simulink model "full_sys"  (R2020a)
settings: Solver=VariableStepAuto  StartTime=0.0  StopTime=0.5  RelTol=1e-3
undefined symbols (not defined in the file): Ion, Lithium
libraries: powerlib x22, simulink x2, electricdrivelib x1
settings Model: EnablePacing=on  PacingRate=10  Creator=siddyq  LastModifiedBy=siddyq

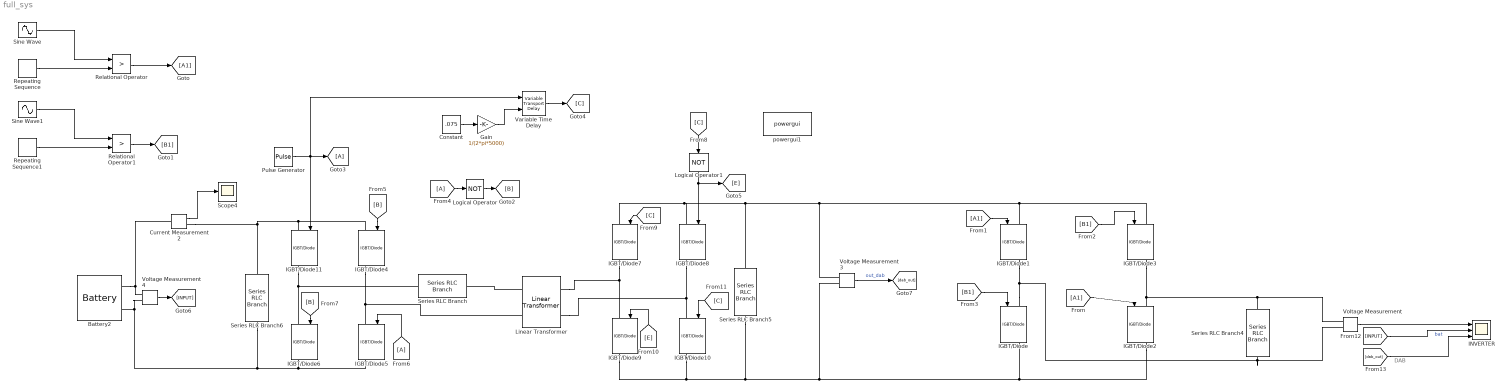
== system full_sys ==
  note: DAB
  Battery2 : electricdrivelib/Extra Sources/Battery  BatType=Lithium-Ion  ShowTempParam=off  ThermalPreset=no  ShowAgeParam=off  NomV=75  NomQ=100  SOC=100  Batt_Tr=1  PresetModel=on  MaxQ=100  MinV=56.25  FullV=87.299  Dis_rate=43.4783  R=0.0075  Normal_OP=90.4348  expZone="[81.0289      4.91304]"  current=[6.5 13 32.5]  Units=Time  Tci=20  NomT=20  T2=-30  MaxQ2=4.8  FullV2=7.1  Normal_OP2=5.655  expZone2="[6.58           1]"  Rca=0.6  ti=2000  Dp=0  Neq0=0  Tsim=1e6  Ta1=25  Qeol=5.4*0.9  Reol=0.013333*1.2  Char_age=[2.3478, 3]  Dis_age=[2.3478, 10]  N1=1500  N2=10500  N3=1000  N4=1400  Ta2=45  N5=950
  Constant : Constant  Value=.075
  Current Measurement2 : powerlib/Measurements/Current Measurement  PhasorSimulation=off  OutputType=Complex  PSBequivalent=0
  Gain : Gain  Gain=1/(2*pi*5000)
  IGBT/Diode{,1..11} (12 alike) : powerlib/Power Electronics/IGBT//Diode  Ron=1e-3  Rs=1e5  Cs=inf  Measurements=on
  INVERTER : Scope  NumInputPorts=3
  Linear Transformer : powerlib/Elements/Linear Transformer  UNITS=SI  NominalPower=[2e2 10000 ]  winding1=[75 0 0]  winding2=[100 0 0]  ThreeWindings=off  winding3=[3.15e+05 66150 42.112]  RmLm=[85555 1.3]  Measurements=None  DataType=on
  Logical Operator : Logic  Operator=NOT  AllPortsSameDT=off  OutDataTypeStr=boolean
  Logical Operator1 : Logic  Operator=NOT  AllPortsSameDT=off  OutDataTypeStr=boolean
  Pulse Generator : DiscretePulseGenerator  PulseType=Time based  Period=1/(2*pi*5000)  PulseWidth=50
  Relational Operator : RelationalOperator  Operator=>  OutDataTypeStr=boolean  RndMeth=Simplest
  Relational Operator1 : RelationalOperator  Operator=>  OutDataTypeStr=boolean  RndMeth=Simplest
  Repeating Sequence : simulink/Sources/Repeating Sequence  rep_seq_t=[0 0.02/40 0.02/20]  rep_seq_y=[0 1 0]
  Repeating Sequence1 : simulink/Sources/Repeating Sequence  rep_seq_t=[0 0.02/40 0.02/20]  rep_seq_y=[0 1 0]
  Scope4 : Scope
  Series RLC Branch : powerlib/Elements/Series RLC Branch  LConnTagsString=__new0  RConnTagsString=__new0  BranchType=L  Resistance=1  Inductance=130e-7  SetiL0=off  InitialCurrent=0  Capacitance=1e-6  Setx0=off  InitialVoltage=0  Measurements=None
  Series RLC Branch4 : powerlib/Elements/Series RLC Branch  LConnTagsString=__new0  RConnTagsString=__new0  BranchType=R  Resistance=10  Inductance=10e-3  SetiL0=off  InitialCurrent=0  Capacitance=1e-6  Setx0=off  InitialVoltage=0  Measurements=None
  Series RLC Branch5 : powerlib/Elements/Series RLC Branch  LConnTagsString=__new0  RConnTagsString=__new0  BranchType=C  Resistance=1  Inductance=1e-3  SetiL0=off  InitialCurrent=0  Capacitance=3000e-6  Setx0=off  InitialVoltage=0  Measurements=None
  Series RLC Branch6 : powerlib/Elements/Series RLC Branch  LConnTagsString=__new0  RConnTagsString=__new0  BranchType=C  Resistance=1  Inductance=1e-3  SetiL0=off  InitialCurrent=0  Capacitance=350e-6  Setx0=off  InitialVoltage=0  Measurements=None
  Sine Wave : Sin  Frequency=100*pi  SampleTime=0
  Sine Wave1 : Sin  Frequency=100*pi  Phase=pi  SampleTime=0
  Variable Time Delay : VariableTransportDelay  MaximumDelay=10  ZeroDelay=on
  Voltage Measurement : powerlib/Measurements/Voltage Measurement  PhasorSimulation=off  OutputType=Complex  PSBequivalent=0
  Voltage Measurement3 : powerlib/Measurements/Voltage Measurement  PhasorSimulation=off  OutputType=Complex  PSBequivalent=0
  Voltage Measurement4 : powerlib/Measurements/Voltage Measurement  PhasorSimulation=off  OutputType=Complex  PSBequivalent=0
  powergui1 : powerlib/powergui  Priority=1  SimulationMode=Discrete  SampleTime=1e-6  frequency=60  Iterations=50  frequencyindice=0  Pbase=100e6  ErrMax=1e-4  UnitsV=kV  UnitsW=MW  buscounter=0  FunctionMessages=off  echomessages=off  EnableUseOfTLC=off  CurrentSourceSwitches=off  DisableSnubberDevices=off  DisableRonSwitches=off  DisableVfSwitches=off  DisplayEquations=off  AutomaticDiscreteSolvers=off  SolverType=Tustin/Backward Euler (TBE)  Interpol=off  ExternalGateDelay=off  methode=off  Ts=100  x0status=blocks  SPID=on  SwTol=0  HookPort=off  NonlinearTolerance=1e-4  nMaxIteration=100  ContinueOnMaxIteration=off  RestoreLinks=warning  ResistiveCurrentMeasurement=off  Frange=[0:2:500]  Ylog=off  Xlog=on  ShowGrid=off  save=off  variable=ZData  structure=0  ZoomFFT=off  StartTime=0.0  cycles=1  DisplayStyle=1  fundamental=60  FreqAxis=off  MaxFrequency=1000  frequencyindicesteady=1  RmsSteady=1  display=off
  wires:
  Relational Operator/1 -> [A1]
  Sine Wave1/1 -> Relational Operator1/1
  Relational Operator1/1 -> [B1]
  Repeating Sequence1/1 -> Relational Operator1/2
  Voltage Measurement/1 -> INVERTER/1
  [A1] -> IGBT/Diode1/1
  [B1] -> IGBT/Diode/1
  [A1] -> IGBT/Diode2/1
  Repeating Sequence/1 -> Relational Operator/2
  Sine Wave/1 -> Relational Operator/1
  [B1] -> IGBT/Diode3/1
  Logical Operator/1 -> [B]
  Voltage Measurement4/1 -> [INPUT]
  [C] -> Logical Operator1/1
  [C] -> IGBT/Diode7/1
  [C] -> IGBT/Diode10/1
  [E] -> IGBT/Diode9/1
  [A] -> IGBT/Diode5/1
  Variable Time Delay/1 -> [C]
  Constant/1 -> Gain/1
  [B] -> IGBT/Diode4/1
  Logical Operator1/1 -> [E], IGBT/Diode8/1
  Voltage Measurement3/1 -> [dab_out]  "out_dab"
  Pulse Generator/1 -> [A], Variable Time Delay/1, IGBT/Diode11/1
  Gain/1 -> Variable Time Delay/2
  [B] -> IGBT/Diode6/1
  [A] -> Logical Operator/1
  [INPUT] -> INVERTER/2  "bat"
  [dab_out] -> INVERTER/3
  Current Measurement2/1 -> Scope4/1
  connections:
  IGBT/Diode/LConn1 -- IGBT/Diode1/RConn1 -- Voltage Measurement/LConn2 -- Series RLC Branch4/LConn1
  Series RLC Branch5/LConn1 -- IGBT/Diode3/LConn1 -- IGBT/Diode1/LConn1 -- Voltage Measurement3/LConn1 -- IGBT/Diode8/LConn1 -- IGBT/Diode7/LConn1
  IGBT/Diode9/RConn1 -- IGBT/Diode10/RConn1 -- Series RLC Branch5/RConn1 -- IGBT/Diode/RConn1 -- IGBT/Diode2/RConn1 -- Voltage Measurement3/LConn2
  Series RLC Branch4/RConn1 -- Voltage Measurement/LConn1 -- IGBT/Diode3/RConn1 -- IGBT/Diode2/LConn1
  IGBT/Diode4/LConn1 -- Current Measurement2/RConn1 -- Series RLC Branch6/LConn1 -- IGBT/Diode11/LConn1
  Linear Transformer/RConn1 -- IGBT/Diode7/RConn1 -- IGBT/Diode9/LConn1
  Linear Transformer/RConn2 -- IGBT/Diode10/LConn1 -- IGBT/Diode8/RConn1
  IGBT/Diode5/RConn1 -- Voltage Measurement4/LConn2 -- Battery2/LConn2 -- Series RLC Branch6/RConn1 -- IGBT/Diode6/RConn1
  IGBT/Diode6/LConn1 -- Series RLC Branch/LConn1 -- IGBT/Diode11/RConn1
  Linear Transformer/LConn2 -- IGBT/Diode5/LConn1 -- IGBT/Diode4/RConn1
  Linear Transformer/LConn1 -- Series RLC Branch/RConn1
  Battery2/LConn1 -- Voltage Measurement4/LConn1 -- Current Measurement2/LConn1
